simulink model "three_phase_voltage_with_frt_emulator_mfcn"  (R2026b)
settings: Solver=VariableStepAuto
undefined symbols (not defined in the file): param
settings Model: Creator=pwr-control  LastModifiedBy=d.bagnara

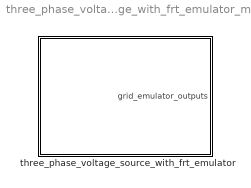
== system three_phase_voltage_with_frt_emulator_mfcn ==
  three_phase_voltage_source_with_frt_emulator : Subsystem  mask(Three-phase voltage emulator with FRT (MATLAB Function)){nominal_frequency_m=param.grid.emu.fgrid_nom, nominal_voltage_m=param.grid.emu.us_secondary_nom, Vemu_ref_norm_m=param.grid.emu.Vemu_ref_norm, vp_xi_pu_m=param.grid.emu.up_xi_pu_ref, vp_eta_pu_m=param.grid.emu.up_eta_pu_ref, vn_xi_pu_m=param.grid.emu.un_xi_pu_ref, vn_eta_pu_m=param.grid.emu.un_eta_pu, Am=param.grid.filters.afe.SOF_50Hz.ss_c.A, Bm=param.grid.filters.afe.SOF_50Hz.ss_c.B, Cm=param.grid.filters.afe.SOF_50Hz.ss_c.C, enable_frt_1_m=param.grid.frt_data.enable_frt_1, enable_frt_2_m=param.grid.frt_data.enable_frt_2, start_time_LVRT_m=param.grid.frt_data.start_time_LVRT, end_time_LVRT_m=param.grid.frt_data.end_time_LVRT, deepPOSxi_m=param.grid.frt_data.deepPOSxi, deepPOSeta_m=param.grid.frt_data.deepPOSeta, deepNEGxi_m=param.grid.frt_data.deepNEGxi, deepNEGeta_m=param.grid.frt_data.deepNEGeta, Amplitude_U_m=param.grid.frt_data.Amplitude_U, Amplitude_V_m=param.grid.frt_data.Amplitude_V, Amplitude_W_m=param.grid.frt_data.Amplitude_W, t_ramp_m=param.grid.frt_data.t_ramp, Phase_shift_m=param.grid.frt_data.Phase_shift}
      mask prompts: nominal_frequency_m "Nominal Frequency [Hz]"; nominal_voltage_m "Nominal Voltage [V]"; Vemu_ref_norm_m "Vemu_ref_norm"; vp_xi_pu_m "Vp_xi_pu [pu]"; vp_eta_pu_m "Vp_eta_pu [pu]"; vn_xi_pu_m "Vn_xi_pu [pu]"; vn_eta_pu_m "Vn_eta_pu [pu]"; Am "LVRT_flt_ss.A"; Bm "LVRT_flt_ss.B"; Cm "LVRT_flt_ss.C"; enable_frt_1_m "enable_frt_1"; enable_frt_2_m "enable_frt_2"; start_time_LVRT_m "Start_time_LVRT"; end_time_LVRT_m "End_time_LVRT"; deepPOSxi_m "deepPOSxi"; deepPOSeta_m "deepPOSeta"; deepNEGxi_m "deepNEGxi"; deepNEGeta_m "deepNEGeta"; Amplitude_U_m "Amplitude_U"; Amplitude_V_m "Amplitude_V"; Amplitude_W_m "Amplitude_W"; t_ramp_m "t_ramp"; Phase_shift_m "Phase_shift"
      mask help:
      | Copy of three_phase_voltage_with_frt_emulator/three_phase_voltage_source_with_frt_emulator written as one MATLAB Function block: same parameters, same output bus grid_emulator_outputs (ua_grid_emu, ub_grid_emu, uc_grid_emu, gamma_grid_emulator, omega_grid_emulator, vp_xi, vp_eta, vn_xi, vn_eta).
      |
      | Steps, rate limiters and variants are written as functions of the simulation time; the eight LVRT filters (A, B, C) keep their continuous states in the Integrator next to the function. 4 non-virtual blocks (the original has 123). The simulation must start at t = 0; enable_frt_1 and enable_frt_2 cannot be both 1.
      mask init:
      | % MATLAB Function copy of three_phase_voltage_with_frt_emulator: checks of the parameters
      | if enable_frt_1_m == 1 && enable_frt_2_m == 1
      |     error(['enable_frt_1 and enable_frt_2 cannot be both 1: the original block has ', ...
      |            'two active variants in that case.']);
      | end
      | nflt = size(Am, 1);
      | if size(Am, 2) ~= nflt || ~isequal(size(Bm), [nflt 1]) || ~isequal(size(Cm), [1 nflt])
      |     error('LVRT_flt_ss: A must be n x n, B n x 1 and C 1 x n (single-input single-output filter).');
      | end
      mask Help: web('https://github.com/pwr-control/library/blob/dev/library/masked_models/power_supply_emulators/README.md', '-browser')
      mask Display:
      | disp(sprintf('three-phase voltage\nemulator with FRT\nMATLAB Function'))
      | port_label('output', 1, 'out')

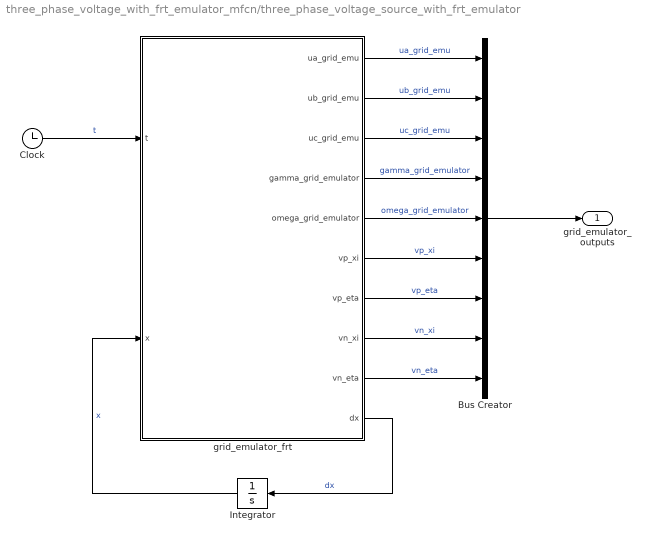
== system three_phase_voltage_with_frt_emulator_mfcn/three_phase_voltage_source_with_frt_emulator ==
  Bus Creator : BusCreator  Inputs=9
  Clock : Clock
  Integrator : Integrator  InitialCondition=zeros(8*size(Am, 1), 1)
  grid_emulator_frt : MATLAB Function  TreatAsAtomicUnit=on
  grid_emulator_outputs : Outport  VectorParamsAs1DForOutWhenUnconnected=off
  wires:
  Clock/1 -> grid_emulator_frt/1(t)  "t"
  grid_emulator_frt/1(ua_grid_emu) -> Bus Creator/1  "ua_grid_emu"
  grid_emulator_frt/2(ub_grid_emu) -> Bus Creator/2  "ub_grid_emu"
  grid_emulator_frt/3(uc_grid_emu) -> Bus Creator/3  "uc_grid_emu"
  grid_emulator_frt/4(gamma_grid_emulator) -> Bus Creator/4  "gamma_grid_emulator"
  grid_emulator_frt/5(omega_grid_emulator) -> Bus Creator/5  "omega_grid_emulator"
  grid_emulator_frt/6(vp_xi) -> Bus Creator/6  "vp_xi"
  grid_emulator_frt/7(vp_eta) -> Bus Creator/7  "vp_eta"
  grid_emulator_frt/8(vn_xi) -> Bus Creator/8  "vn_xi"
  grid_emulator_frt/9(vn_eta) -> Bus Creator/9  "vn_eta"
  Bus Creator/1 -> grid_emulator_outputs/1
  grid_emulator_frt/10(dx) -> Integrator/1  "dx"
  Integrator/1 -> grid_emulator_frt/2(x)  "x"

== matlab function three_phase_voltage_with_frt_emulator_mfcn/three_phase_voltage_source_with_frt_emulator/grid_emulator_frt ==
  data: t input; x input; ua_grid_emu output; ub_grid_emu output; uc_grid_emu output; gamma_grid_emulator output; omega_grid_emulator output; vp_xi output; vp_eta output; vn_xi output; vn_eta output; dx output; nominal_frequency_m parameter; nominal_voltage_m parameter; Vemu_ref_norm_m parameter; vp_xi_pu_m parameter; vp_eta_pu_m parameter; vn_xi_pu_m parameter; vn_eta_pu_m parameter; Am parameter; Bm parameter; Cm parameter; enable_frt_1_m parameter; enable_frt_2_m parameter; start_time_LVRT_m parameter; end_time_LVRT_m parameter; deepPOSxi_m parameter; deepPOSeta_m parameter; deepNEGxi_m parameter; deepNEGeta_m parameter; Amplitude_U_m parameter; Amplitude_V_m parameter; Amplitude_W_m parameter; t_ramp_m parameter; Phase_shift_m parameter
function [ua_grid_emu, ub_grid_emu, uc_grid_emu, gamma_grid_emulator, omega_grid_emulator, ...
    vp_xi, vp_eta, vn_xi, vn_eta, dx] = grid_emulator_frt(t, x, ...
    nominal_frequency_m, nominal_voltage_m, Vemu_ref_norm_m, ...
    vp_xi_pu_m, vp_eta_pu_m, vn_xi_pu_m, vn_eta_pu_m, Am, Bm, Cm, ...
    enable_frt_1_m, enable_frt_2_m, start_time_LVRT_m, end_time_LVRT_m, ...
    deepPOSxi_m, deepPOSeta_m, deepNEGxi_m, deepNEGeta_m, ...
    Amplitude_U_m, Amplitude_V_m, Amplitude_W_m, t_ramp_m, Phase_shift_m)
%#codegen
% GRID_EMULATOR_FRT
% MATLAB Function copy of three_phase_voltage_with_frt_emulator/
% three_phase_voltage_source_with_frt_emulator: same mask parameters, same output bus.
% The Step, Rate Limiter, Constant, Sum and MATLAB Function blocks of the original are
% written here as functions of the time t. The eight LVRT state-space filters
% (Am, Bm, Cm) keep their continuous states: they are integrated by the Integrator
% block next to this function, which receives dx and returns x.
%
% INPUTS
%   t : simulation time [s], from the Clock block (the simulation must start at t = 0)
%   x : states of the eight LVRT filters, 8*size(Am,1) x 1, zero at t = 0.
%       Filter k uses x((k-1)*n+1 : k*n), n = size(Am,1):
%       1 vp_xi, 2 vp_eta, 3 vn_xi, 4 vn_eta  (sequence references [pu])
%       5, 6, 7 amplitudes of the phases U, V, W [pu], 8 phase shift [rad]
%
% PARAMETERS: the 23 mask parameters of the block, in the order of the mask (arguments
%   with scope Parameter, no ports)
%
% OUTPUTS (elements of the bus grid_emulator_outputs, same order as the original)
%   ua_grid_emu, ub_grid_emu, uc_grid_emu : phase voltages [V]
%   gamma_grid_emulator : grid angle, wrapped to [-pi, pi) [rad]
%   omega_grid_emulator : grid angular frequency [rad/s]
%   vp_xi, vp_eta, vn_xi, vn_eta : filtered sequence voltages [V]
%   dx : derivative of x, to the Integrator
%
% VARIANTS (the Variant Source blocks of the original, same conditions)
%   enable_frt_1_m = 0, enable_frt_2_m = 0 : constant sequence references
%   enable_frt_2_m = 1 : dips on the sequence references (deep* parameters)
%   enable_frt_1_m = 1 : dips on the phase amplitudes (Amplitude_U/V/W) and phase
%                        shift of V and W; the sequence outputs follow the deep* profile
%   The two flags cannot be both 1 (two active variants in the original): the mask
%   initialization stops with an error.

n    = size(Am, 1);
kv   = nominal_voltage_m/sqrt(3/2);      % Gain blocks [V/pu]
vref = Vemu_ref_norm_m;
slew = Vemu_ref_norm_m/t_ramp_m;         % Rate Limiters: rising +slew, falling -slew [pu/s]
ton  = start_time_LVRT_m;
toff = end_time_LVRT_m;

frt_seq = (enable_frt_1_m || enable_frt_2_m);   % voltage_source: (enable_frt_1 || enable_frt_2) == 1
frt_abc = (enable_frt_1_m == 1);                % voltage_reference1: enable_frt_1 == 1

% phase_gen1: Constant -> Integrator (starts from 0) -> bounder
omega_grid_emulator = nominal_frequency_m*2*pi;
gamma_grid_emulator = -pi + mod(omega_grid_emulator*t + 3*pi, 2*pi);

% inputs of the eight filters
u = zeros(8, 1);
if frt_seq
    % voltage_source: Step at 0, start, end -> Rate Limiter -> Add (+ - +)
    dp_xi = vp_xi_pu_m*deepPOSxi_m;
    u(1) = rl_step(t, 0, vp_xi_pu_m, slew) - rl_step(t, ton, dp_xi, slew) ...
         + rl_step(t, toff, dp_xi, slew);
    u(2) = rl_step(t, 0, vp_eta_pu_m, slew) - rl_step(t, ton, deepPOSeta_m, slew) ...
         + rl_step(t, toff, deepPOSeta_m, slew);
    u(3) = rl_step(t, 0, vn_xi_pu_m, slew) - rl_step(t, ton, deepNEGxi_m, slew) ...
         + rl_step(t, toff, deepNEGxi_m, slew);
    u(4) = rl_step(t, 0, vn_eta_pu_m, slew) - rl_step(t, ton, deepNEGeta_m, slew) ...
         + rl_step(t, toff, deepNEGeta_m, slew);
else
    % voltage_source: Constant blocks
    u(1) = vp_xi_pu_m;
    u(2) = vp_eta_pu_m;
    u(3) = vn_xi_pu_m;
    u(4) = vn_eta_pu_m;
end
if frt_abc
    % voltage_source_with_frt: Step at 0, start, end -> Rate Limiter -> Add (+ - +) for
    % each phase; phase shift: Step at start - Step at end, without Rate Limiter
    du = vref*(1 - Amplitude_U_m);
    dv = vref*(1 - Amplitude_V_m);
    dw = vref*(1 - Amplitude_W_m);
    u(5) = rl_step(t, 0, vref, slew) - rl_step(t, ton, du, slew) + rl_step(t, toff, du, slew);
    u(6) = rl_step(t, 0, vref, slew) - rl_step(t, ton, dv, slew) + rl_step(t, toff, dv, slew);
    u(7) = rl_step(t, 0, vref, slew) - rl_step(t, ton, dw, slew) + rl_step(t, toff, dw, slew);
    u(8) = Phase_shift_m*step_at(t, ton) - Phase_shift_m*step_at(t, toff);
end

% ss_flt: dx/dt = Am*x + Bm*u, y = Cm*x (no D term, as in the original)
xc = x(:);
dx = zeros(8*n, 1);
y  = zeros(8, 1);
for k = 1:8
    idx = (k - 1)*n + (1:n);
    xk = xc(idx);
    dx(idx) = Am*xk + Bm*u(k);
    y(k) = Cm*xk;
end

% Gain nominal_voltage_m/sqrt(3/2)
vp_xi  = kv*y(1);
vp_eta = kv*y(2);
vn_xi  = kv*y(3);
vn_eta = kv*y(4);

if frt_abc
    % voltage_source_with_frt: Phase_a1, Phase_b1, Phase_c1, then Gain
    ua_grid_emu = kv*(y(5)*cos(gamma_grid_emulator));
    ub_grid_emu = kv*(y(6)*cos(gamma_grid_emulator - y(8) - 2*pi/3));
    uc_grid_emu = kv*(y(7)*cos(gamma_grid_emulator + y(8) - 4*pi/3));
else
    % voltage_reference1: xieta2alphabeta_pos + xieta2alphabeta_neg -> alphabeta2abc
    c = cos(gamma_grid_emulator);
    s = sin(gamma_grid_emulator);
    alpha = (vp_xi*c - vp_eta*s) + (vn_xi*c + vn_eta*s);
    beta  = (vp_xi*s + vp_eta*c) + (-vn_xi*s + vn_eta*c);
    ua_grid_emu = alpha;
    ub_grid_emu = -0.5*alpha + sqrt(3)/2*beta;
    uc_grid_emu = -0.5*alpha - sqrt(3)/2*beta;
end
end

function y = step_at(t, t_step)
% Step block: 0 before t_step, 1 from t_step on
y = 0;
if t >= t_step
    y = 1;
end
end

function y = rl_step(t, t_step, v, slew)
% Step block (0 -> v at t_step) followed by a continuous-time Rate Limiter with rising
% slew rate +slew and falling slew rate -slew. In continuous mode the Rate Limiter
% starts from its input (y(0) = u(0)), so a step at t = 0 passes without ramp; a later
% step becomes a ramp of slope slew that ends on v.
y = 0;
if t >= t_step
    if t_step <= 0 || ~(slew < Inf)
        y = v;
    else
        r = slew*(t - t_step);
        if r >= abs(v)
            y = v;
        elseif v >= 0
            y = r;
        else
            y = -r;
        end
    end
end
end
